simulink model "emso_uotr"  (Simulink 7.1)
settings: Solver=ode45  StartTime=0.0  StopTime=3600  RelTol=1e-3
settings Model: Creator=lades  LastModifiedBy=W7
settings DataIOCC: ExternalInput=Az
settings DebuggingCC: SaveWithDisabledLinksMsg=none  SaveWithParameterizedLinksMsg=none  CheckSSInitialOutputMsg=off  SolverPrmCheckMsg=none  MultiTaskCondExecSysMsg=none  Int32ToFloatConvMsg=none  ModelReferenceDataLoggingMessage=none

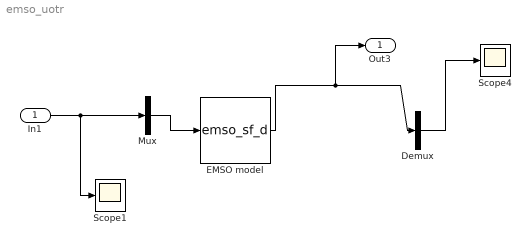
== system emso_uotr ==
  In1 : Inport
  Demux : Demux  Outputs=1
  EMSO model : S-Function  FunctionName=emso_sf_d  Parameters='emso_uotr.ems',2,1,0.5  EnableBusSupport=off
  Mux : Mux  Inputs=1
  Scope1 : Scope
      settings: TimeRange=2  YMin=4.008258966500001  YMax=4.008258969500001
  Scope4 : Scope
      settings: TimeRange=5  YMin=0  YMax=45  SaveName=ScopeData3
  Out3 : Outport
  wires:
  EMSO model/1 -> Demux/1, Out3/1
  Mux/1 -> EMSO model/1
  In1/1 -> Mux/1, Scope1/1
  Demux/1 -> Scope4/1
